simulink model "PiSOCAIReference"  (R2026b)
settings: Solver=FixedStepDiscrete  FixedStep=1  EnableMultiTasking=on
values from neighbouring files (symbols this model uses):
  biasIn : value not decoded    [main_LSTM.sldd]
  biasOut = 0.22654434469969603    [main_LSTM.sldd]
  scalerIn : value not decoded    [main_LSTM.sldd]
  scalerOut = 0.69775663669108012    [main_LSTM.sldd]
libraries: deeplib x1
settings Model: Creator=mgado  LastModifiedBy=mgado
settings SolverCC: PositivePriorityOrder=on
settings DataIOCC: SaveOutput=off  SaveTime=off
settings OptimizationCC: DifferentSizesBufferReuse=on  EfficientTunableParamExpr=on  EnhancedBackFolding=on  MaxStackSize=200000  OptimizationCustomize=off  OptimizeBlockOrder=speed  PassReuseOutputArgsAs=Individual arguments  RemoveInternalMemoryZeroInit=on  RemoveRootLevelIOMemoryZeroInit=on
settings DebuggingCC: ParameterTunabilityLossMsg=error
settings HardwareCC: ProdHWDeviceType=ARM Compatible->ARM Cortex-A (32-bit)  ProdLargestAtomicFloat=Double  ProdLargestAtomicInteger=Long  ProdLongLongMode=on
settings ModelReferenceCC: PropagateVarSize=During execution
settings RTWCC: BuildConfiguration=Faster Runs  Description=Embedded Coder  GPUComputeCapability=5.0  HardwareBoard=Raspberry Pi  SystemTargetFile=ert.tlc  TLCOptions="-aInlineSetEventsForThisBaseRateFcn=TLC_FALSE -aSuppressMultiTaskScheduler=TLC_FALSE  -aRateBasedStepFcn=0"  TemplateMakefile=ert_default_tmf  Toolchain=GNU GCC RPIUtils
settings CodeAppCC: ForceParamTrailComments=on  IgnoreCustomStorageClasses=off  InsertBlockDesc=on  OperatorAnnotations=on  SFDataObjDesc=on  SimulinkDataObjDesc=on
settings ERTTargetCC: ExtModeIntrfLevel=Level2 - Open  ExtModeMexFile=ext_xcp  ExtModeStaticAlloc=on  SupportVariableSizeSignals=on

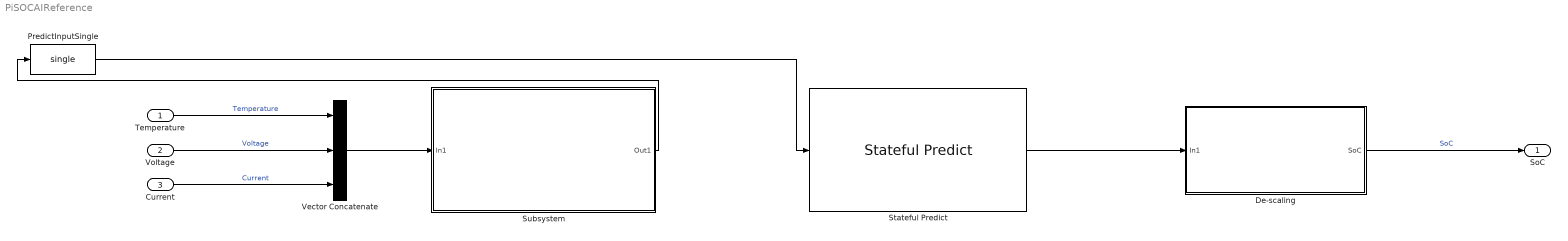
== system PiSOCAIReference ==
  Temperature : Inport
  Voltage : Inport  Port=2
  Current : Inport  Port=3
  De-scaling : Subsystem
  PredictInputSingle : DataTypeConversion  OutDataTypeStr=single  SaturateOnIntegerOverflow=off  RndMeth=Floor
  Stateful Predict : deeplib/Stateful Predict  Network=Network from MAT-file  NetworkFunction=untitled  NetworkFilePath=projected_net.mat  NetworkWorkspaceVariable=net  SimulateUsing=Auto mode  InputDataFormats={'input_layer', 'CT';}  SampleTime=-1  ForceInterpretedSim=off  EnableDLNetwork=on  LastKnownNetworkFilePath='projected_net.mat'  LastKnownNetworkTimeStamp=740302.566250000032596290111541748046875
  Subsystem : Subsystem
  Vector Concatenate : Concatenate  NumInputs=3  Mode=Multidimensional array
  SoC : Outport
  wires:
  De-scaling/1(SoC) -> SoC/1  "SoC"
  Voltage/1 -> Vector Concatenate/2  "Voltage"
  Current/1 -> Vector Concatenate/3  "Current"
  Temperature/1 -> Vector Concatenate/1  "Temperature"
  Stateful Predict/1 -> De-scaling/1(In1)
  Vector Concatenate/1 -> Subsystem/1(In1)
  Subsystem/1(Out1) -> PredictInputSingle/1
  PredictInputSingle/1 -> Stateful Predict/1

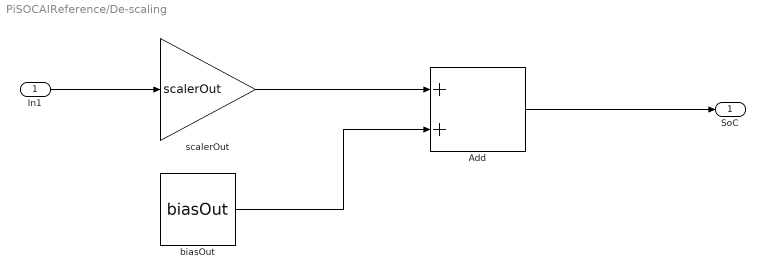
== system PiSOCAIReference/De-scaling ==
  In1 : Inport
  Add : Sum
  biasOut : Constant  Value=biasOut
  scalerOut : Gain  Gain=scalerOut
  SoC : Outport
  wires:
  In1/1 -> scalerOut/1
  scalerOut/1 -> Add/1
  biasOut/1 -> Add/2
  Add/1 -> SoC/1

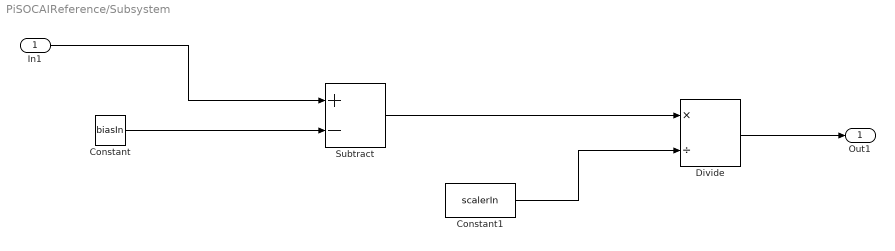
== system PiSOCAIReference/Subsystem ==
  In1 : Inport
  Constant : Constant  Value=biasIn
  Constant1 : Constant  Value=scalerIn
  Divide : Product  Inputs=*/
  Subtract : Sum  Inputs=+-
  Out1 : Outport
  wires:
  Subtract/1 -> Divide/1
  Divide/1 -> Out1/1
  Constant/1 -> Subtract/2
  In1/1 -> Subtract/1
  Constant1/1 -> Divide/2
